simulink model "ACC_Stage43GE_Experimental"  (R2025b)
settings: Solver=ode45  StartTime=0.0  StopTime=60  MaxStep=0.05  RelTol=1e-3
PreLoadFcn:
  | init_workspace;
InitFcn:
  | if ~exist('x0', 'var'), init_workspace; end;
undefined symbols (not defined in the file): K_tube_active, stage45_mpc_dispatcher, t_gust_off, t_gust_on, Ts, x0
settings Model: Creator=avina  LastModifiedBy=avina

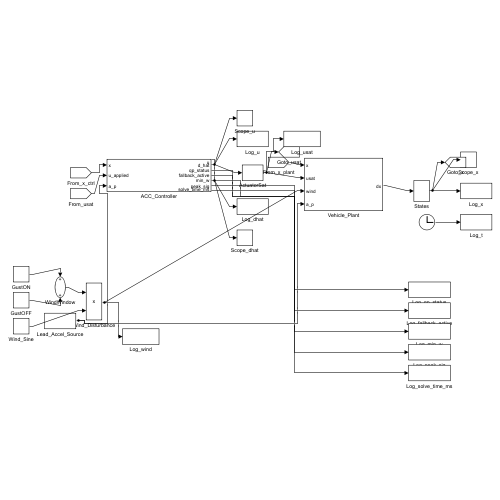
[thumbnail: Simulink's stored preview of the top-level diagram]
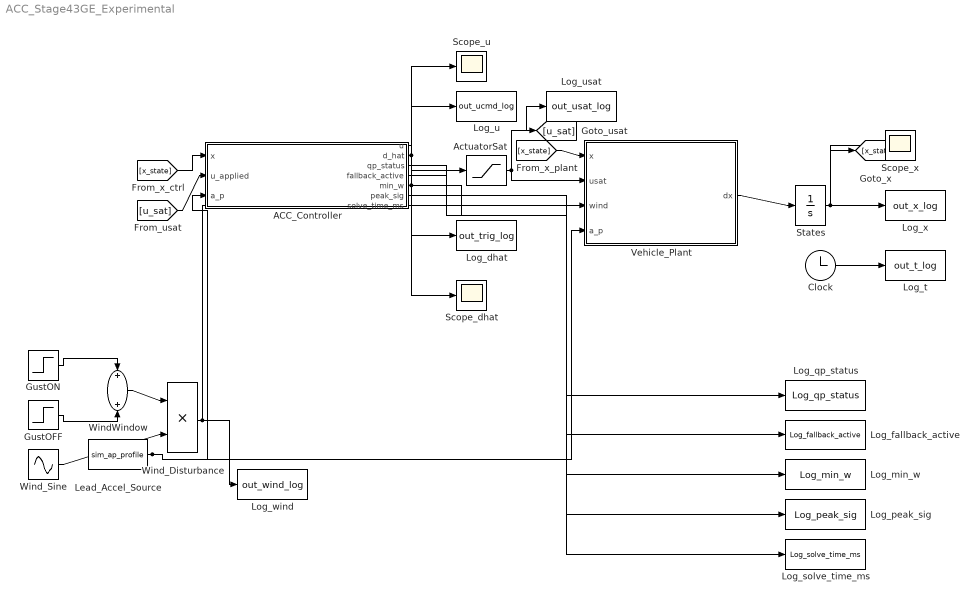
== system ACC_Stage43GE_Experimental ==
  ACC_Controller : Subsystem
  ActuatorSat : Saturate  UpperLimit=2.5  LowerLimit=-3
  Clock : Clock
  GustOFF : Step  Time=t_gust_off  After=-1  SampleTime=0
  GustON : Step  Time=t_gust_on  SampleTime=0
  Lead_Accel_Source : FromWorkspace  VariableName=sim_ap_profile
  Log_dhat : ToWorkspace  VariableName=out_trig_log  SampleTime=-1
  Log_fallback_active : ToWorkspace  VariableName=Log_fallback_active  SampleTime=Ts
  Log_min_w : ToWorkspace  VariableName=Log_min_w  SampleTime=Ts
  Log_peak_sig : ToWorkspace  VariableName=Log_peak_sig  SampleTime=Ts
  Log_qp_status : ToWorkspace  VariableName=Log_qp_status  SampleTime=Ts
  Log_solve_time_ms : ToWorkspace  VariableName=Log_solve_time_ms  SampleTime=Ts
  Log_t : ToWorkspace  VariableName=out_t_log  SampleTime=-1
  Log_u : ToWorkspace  VariableName=out_ucmd_log  SampleTime=-1
  Log_usat : ToWorkspace  VariableName=out_usat_log  SampleTime=-1
  Log_wind : ToWorkspace  VariableName=out_wind_log  SampleTime=0.1
  Log_x : ToWorkspace  VariableName=out_x_log  SampleTime=-1
  Scope_dhat : Scope
  Scope_u : Scope
  Scope_x : Scope
  States : Integrator  InitialCondition=x0
  Vehicle_Plant : Subsystem
  WindWindow : Sum
  Wind_Disturbance : Product
  Wind_Sine : Sin  Amplitude=0.25  Frequency=0.314  SampleTime=0
  wires:
  GustON/1 -> WindWindow/1
  GustOFF/1 -> WindWindow/2
  WindWindow/1 -> Wind_Disturbance/1
  Wind_Sine/1 -> Wind_Disturbance/2
  ACC_Controller/1(u) -> ActuatorSat/1, Log_u/1, Scope_u/1
  ActuatorSat/1 -> Vehicle_Plant/2(usat), [u_sat], Log_usat/1
  Wind_Disturbance/1 -> Vehicle_Plant/3(wind), Log_wind/1
  Vehicle_Plant/1(dx) -> States/1
  Clock/1 -> Log_t/1
  States/1 -> Log_x/1, Scope_x/1, [x_state]
  ACC_Controller/2(d_hat) -> Log_dhat/1, Scope_dhat/1
  [x_state] -> ACC_Controller/1(x)
  [x_state] -> Vehicle_Plant/1(x)
  [u_sat] -> ACC_Controller/2(u_applied)
  Lead_Accel_Source/1 -> Vehicle_Plant/4(a_p), ACC_Controller/3(a_p)
  ACC_Controller/3(qp_status) -> Log_qp_status/1
  ACC_Controller/4(fallback_active) -> Log_fallback_active/1
  ACC_Controller/5(min_w) -> Log_min_w/1
  ACC_Controller/6(peak_sig) -> Log_peak_sig/1
  ACC_Controller/7(solve_time_ms) -> Log_solve_time_ms/1

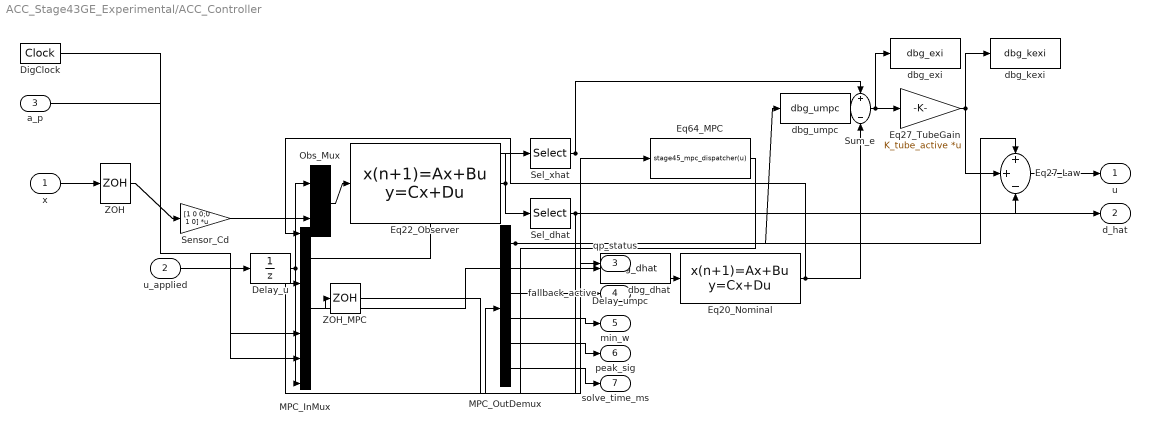
== system ACC_Stage43GE_Experimental/ACC_Controller ==
  x : Inport
  u_applied : Inport  Port=2
  a_p : Inport  Port=3
  Delay_u : UnitDelay  SampleTime=0.1  HasFrameUpgradeWarning=on
  Delay_umpc : UnitDelay  SampleTime=0.1  HasFrameUpgradeWarning=on
  DigClock : DigitalClock  SampleTime=Ts
  Eq20_Nominal : DiscreteStateSpace  A=[1 0.069435 -0.15399;0 0.98007 -0.099335;0 0.39734 0.98007]  B=[-0.015283;-0.0099667;0.19867]  C=[1 0 0;0 1 0;0 0 1]  D=zeros(3,1)  InitialCondition=x0  SampleTime=0.1
  Eq22_Observer : DiscreteStateSpace  A=[-0.16504 -0.1497 -0.15399 -0.0076414;-0.16027 -0.017086 -0.099335 -0.0049834;1.5608 1.0061 0.98007 0.099335;2.0229 1.3025 0 1]  B=[-0.015283 1.165 0.21913;-0.0099667 0.16027 0.99715;0.19867 -1.5608 -0.60878;0 -2.0229 -1.3025]  C=[1 0 0 0;0 1 0 0;0 0 1 0;0 0 0 1]  D=zeros(4,3)  InitialCondition=[x0; 0]  SampleTime=0.1
  Eq27_Law : Sum  Inputs=++-
  Eq27_TubeGain : Gain  Gain=K_tube_active  Multiplication=Matrix(K*u)
  Eq64_MPC : MATLABFcn  MATLABFcn=stage45_mpc_dispatcher(u)  OutputDimensions=6
  MPC_InMux : Mux  Inputs=7
  MPC_OutDemux : Demux  Outputs=6
  Obs_Mux : Mux  Inputs=[1;2]
  Sel_dhat : Selector  InputPortWidth=4  IndexOptions=Index vector (dialog)  Indices=4  OutputSizes=1
  Sel_xhat : Selector  InputPortWidth=4  IndexOptions=Index vector (dialog)  Indices=1:3  OutputSizes=1
  Sensor_Cd : Gain  Gain=[1 0 0;0 1 0]  Multiplication=Matrix(K*u)
  Sum_e : Sum  Inputs=+-
  ZOH : ZeroOrderHold  SampleTime=0.1
  ZOH_MPC : ZeroOrderHold  SampleTime=Ts
  dbg_dhat : ToWorkspace  VariableName=dbg_dhat  SaveFormat=Timeseries  SampleTime=-1
  dbg_exi : ToWorkspace  VariableName=dbg_exi  SaveFormat=Timeseries  SampleTime=-1
  dbg_kexi : ToWorkspace  VariableName=dbg_kexi  SaveFormat=Timeseries  SampleTime=-1
  dbg_umpc : ToWorkspace  VariableName=dbg_umpc  SaveFormat=Timeseries  SampleTime=-1
  u : Outport
  d_hat : Outport  Port=2
  qp_status : Outport  Port=3
  fallback_active : Outport  Port=4
  min_w : Outport  Port=5
  peak_sig : Outport  Port=6
  solve_time_ms : Outport  Port=7
  wires:
  x/1 -> ZOH/1
  ZOH/1 -> Sensor_Cd/1
  Delay_u/1 -> Obs_Mux/1, MPC_InMux/7
  Sensor_Cd/1 -> Obs_Mux/2
  Obs_Mux/1 -> Eq22_Observer/1
  Eq22_Observer/1 -> Sel_xhat/1, Sel_dhat/1
  Sel_xhat/1 -> Sum_e/1, MPC_InMux/2
  Delay_umpc/1 -> Eq20_Nominal/1, MPC_InMux/4
  Eq20_Nominal/1 -> Sum_e/2, MPC_InMux/1
  Sum_e/1 -> Eq27_TubeGain/1, dbg_exi/1
  Eq27_TubeGain/1 -> Eq27_Law/2, dbg_kexi/1
  Sel_dhat/1 -> Eq27_Law/3, d_hat/1, dbg_dhat/1, MPC_InMux/3
  Eq27_Law/1 -> u/1
  u_applied/1 -> Delay_u/1
  a_p/1 -> MPC_InMux/5
  DigClock/1 -> MPC_InMux/6
  Eq64_MPC/1 -> MPC_OutDemux/1
  MPC_OutDemux/1 -> Delay_umpc/1, Eq27_Law/1, dbg_umpc/1
  MPC_OutDemux/2 -> qp_status/1
  MPC_OutDemux/3 -> fallback_active/1
  MPC_OutDemux/4 -> min_w/1
  MPC_OutDemux/5 -> peak_sig/1
  MPC_OutDemux/6 -> solve_time_ms/1
  MPC_InMux/1 -> ZOH_MPC/1
  ZOH_MPC/1 -> Eq64_MPC/1

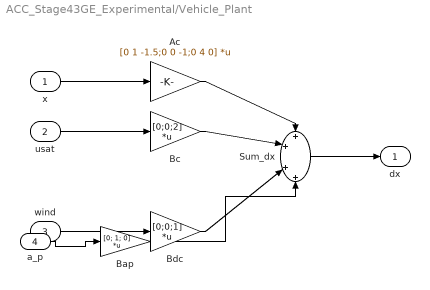
== system ACC_Stage43GE_Experimental/Vehicle_Plant ==
  x : Inport
  usat : Inport  Port=2
  wind : Inport  Port=3
  a_p : Inport  Port=4
  Ac : Gain  Gain=[0 1 -1.5;0 0 -1;0 4 0]  Multiplication=Matrix(K*u)
  Bap : Gain  Gain=[0; 1; 0]  Multiplication=Matrix(K*u)
  Bc : Gain  Gain=[0;0;2]  Multiplication=Matrix(K*u)
  Bdc : Gain  Gain=[0;0;1]  Multiplication=Matrix(K*u)
  Sum_dx : Sum  Inputs=++++
  dx : Outport
  wires:
  x/1 -> Ac/1
  Ac/1 -> Sum_dx/1
  usat/1 -> Bc/1
  Bc/1 -> Sum_dx/2
  wind/1 -> Bdc/1
  Bdc/1 -> Sum_dx/3
  Sum_dx/1 -> dx/1
  a_p/1 -> Bap/1
  Bap/1 -> Sum_dx/4
